simulink library "Batteries"  (R2026a)
settings: Solver=VariableStepAuto
undefined symbols (not defined in the file or in its folder): battery_builder_rtmsupport, gcbh
libraries: Batteries_lib x2
settings Model: Creator=dom  LastModifiedBy=dom

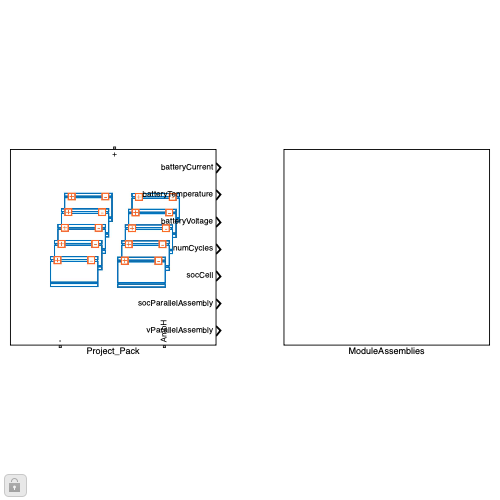
[thumbnail: Simulink's stored preview of the top-level diagram]
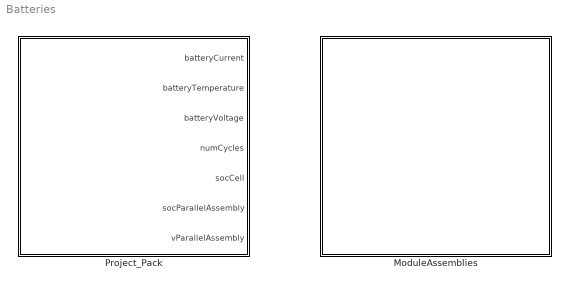
== system Batteries ==
  ModuleAssemblies : Subsystem
  Project_Pack : Subsystem  LoadFcn=battery_builder_rtmsupport('loadfcn',gcbh);
      settings: CopyFcn=battery_builder_rtmsupport('copyfcn',gcbh);  PreCopyFcn=battery_builder_rtmsupport('precopyfcn',gcbh);  PreDeleteFcn=battery_builder_rtmsupport('predeletefcn',gcbh);  PortSchema="{\"entries\":[{\"content\":{\"sides\":[{\"content\":{\"connectorIds\":[\"LConn1\"]},\"type\":\"ConnectorPlacement.EquallySpacedRectSide\",\"uuid\":\"76c6f046-db8e-4015-a922-00ba973faf16\"},{\"content\":{\"connectorIds\":[\"RConn1\",\"RConn2\"],\"side\":\"RIGHT\"},\"type\":\"ConnectorPlacement.EquallySpacedRectSide\",\"uuid\":\"59fdee5c-a6f4-4b44-aa6e-82d2d9418fce\"},{\"content\":{\"side\":\"TOP\"},\"type\":\"ConnectorPlacement.EquallySpacedRectSide\",\"uuid\":\"84b83595-cc1f-46da-a2b0-c16634a6daab\"},{\"content\":{\"connectorIds\":[\"Out1\",\"Out2\",\"Out3\",\"Out4\",\"Out5\",\"Out6\",\"Out7\"],\"side\":\"BOTTOM\"},\"type\":\"ConnectorPlacement.EquallySpacedRectSide\",\"uuid\":\"4528fa0d-8164-4e66-baa6-2a345765de4f\"}]},\"type\":\"ConnectorPlacement.EquallySpacedConnector\",\"uuid\":\"e6fb231a-8daf-4bfc-bdc1-9175fa7a2dfd\"}],\"packageUris\":[\"http://schema.mathworks.com/mf0/Connector/R2020b\"],\"version\":\"1.0\"}"
      mask Display: image('$imagefile')

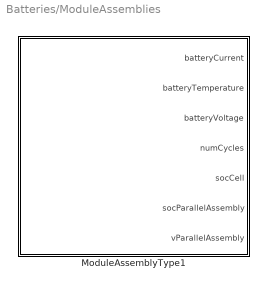
== system Batteries/ModuleAssemblies ==
  ModuleAssemblyType1 : Subsystem  LoadFcn=battery_builder_rtmsupport('loadfcn',gcbh);
      settings: CopyFcn=battery_builder_rtmsupport('copyfcn',gcbh);  PreCopyFcn=battery_builder_rtmsupport('precopyfcn',gcbh);  PreDeleteFcn=battery_builder_rtmsupport('predeletefcn',gcbh);  PortSchema="{\"entries\":[{\"content\":{\"sides\":[{\"content\":{\"connectorIds\":[\"LConn1\"]},\"type\":\"ConnectorPlacement.EquallySpacedRectSide\",\"uuid\":\"76c6f046-db8e-4015-a922-00ba973faf16\"},{\"content\":{\"connectorIds\":[\"RConn1\",\"RConn2\"],\"side\":\"RIGHT\"},\"type\":\"ConnectorPlacement.EquallySpacedRectSide\",\"uuid\":\"59fdee5c-a6f4-4b44-aa6e-82d2d9418fce\"},{\"content\":{\"side\":\"TOP\"},\"type\":\"ConnectorPlacement.EquallySpacedRectSide\",\"uuid\":\"84b83595-cc1f-46da-a2b0-c16634a6daab\"},{\"content\":{\"connectorIds\":[\"Out1\",\"Out2\",\"Out3\",\"Out4\",\"Out5\",\"Out6\",\"Out7\"],\"side\":\"BOTTOM\"},\"type\":\"ConnectorPlacement.EquallySpacedRectSide\",\"uuid\":\"391f6102-8f79-4306-a331-0bb83eeeb4a2\"}]},\"type\":\"ConnectorPlacement.EquallySpacedConnector\",\"uuid\":\"e6fb231a-8daf-4bfc-bdc1-9175fa7a2dfd\"}],\"packageUris\":[\"http://schema.mathworks.com/mf0/Connector/R2020b\"],\"version\":\"1.0\"}"
      mask Display: image('$imagefile')

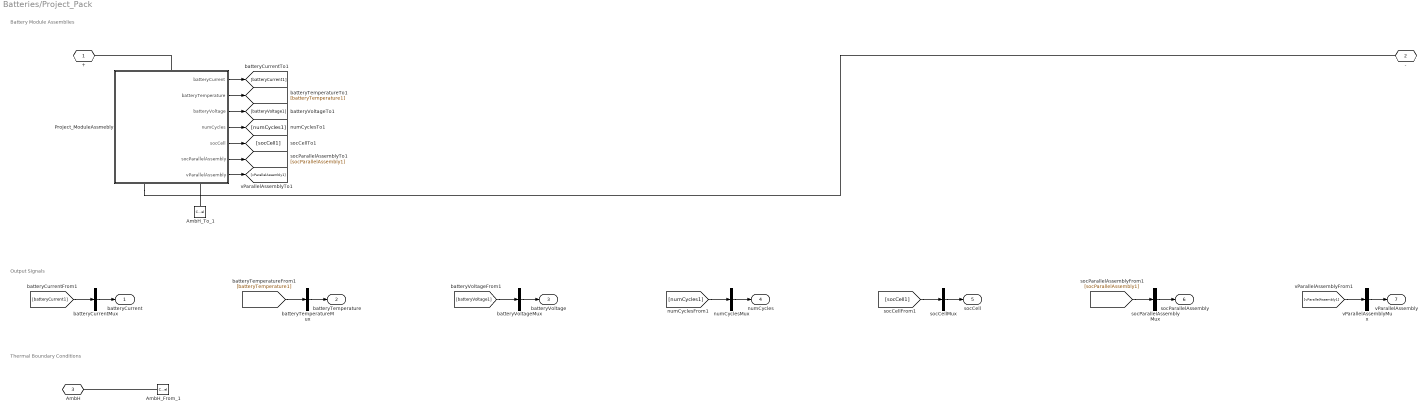
== system Batteries/Project_Pack ==
  note: Battery Module Assemblies
  note: Output Signals
  note: Thermal Boundary Conditions
  AmbH_From_1 : ConnectionLabel  Label=ambH_1
  AmbH_To_1 : ConnectionLabel  Label=ambH_1
  Project_ModuleAssmebly : Subsystem  LoadFcn=battery_builder_rtmsupport('loadfcn',gcbh);
      settings: CopyFcn=battery_builder_rtmsupport('copyfcn',gcbh);  PreCopyFcn=battery_builder_rtmsupport('precopyfcn',gcbh);  PreDeleteFcn=battery_builder_rtmsupport('predeletefcn',gcbh);  PortSchema="{\"entries\":[{\"content\":{\"sides\":[{\"content\":{\"connectorIds\":[\"LConn1\"]},\"type\":\"ConnectorPlacement.EquallySpacedRectSide\",\"uuid\":\"76c6f046-db8e-4015-a922-00ba973faf16\"},{\"content\":{\"connectorIds\":[\"RConn1\",\"RConn2\"],\"side\":\"RIGHT\"},\"type\":\"ConnectorPlacement.EquallySpacedRectSide\",\"uuid\":\"59fdee5c-a6f4-4b44-aa6e-82d2d9418fce\"},{\"content\":{\"side\":\"TOP\"},\"type\":\"ConnectorPlacement.EquallySpacedRectSide\",\"uuid\":\"84b83595-cc1f-46da-a2b0-c16634a6daab\"},{\"content\":{\"connectorIds\":[\"Out1\",\"Out2\",\"Out3\",\"Out4\",\"Out5\",\"Out6\",\"Out7\"],\"side\":\"BOTTOM\"},\"type\":\"ConnectorPlacement.EquallySpacedRectSide\",\"uuid\":\"391f6102-8f79-4306-a331-0bb83eeeb4a2\"}]},\"type\":\"ConnectorPlacement.EquallySpacedConnector\",\"uuid\":\"e6fb231a-8daf-4bfc-bdc1-9175fa7a2dfd\"}],\"packageUris\":[\"http://schema.mathworks.com/mf0/Connector/R2020b\"],\"version\":\"1.0\"}"
      mask Display: image('$imagefile')
  batteryCurrentMux : Mux  Inputs=1
  batteryTemperatureMux : Mux  Inputs=1
  batteryVoltageMux : Mux  Inputs=1
  numCyclesMux : Mux  Inputs=1
  socCellMux : Mux  Inputs=1
  socParallelAssemblyMux : Mux  Inputs=1
  vParallelAssemblyMux : Mux  Inputs=1
  + : PMIOPort  Side=Left
  - : PMIOPort  Port=2  Side=Right
  AmbH : PMIOPort  Port=3  Side=Right  ConnectionType=Connection: foundation.thermal.thermal
  batteryCurrent : Outport
  batteryTemperature : Outport  Port=2
  batteryVoltage : Outport  Port=3
  numCycles : Outport  Port=4
  socCell : Outport  Port=5
  socParallelAssembly : Outport  Port=6
  vParallelAssembly : Outport  Port=7
  wires:
  Project_ModuleAssmebly/1(batteryCurrent) -> [batteryCurrent1]
  batteryCurrentMux/1 -> batteryCurrent/1
  [batteryCurrent1] -> batteryCurrentMux/1
  Project_ModuleAssmebly/2(batteryTemperature) -> [batteryTemperature1]
  batteryTemperatureMux/1 -> batteryTemperature/1
  [batteryTemperature1] -> batteryTemperatureMux/1
  Project_ModuleAssmebly/3(batteryVoltage) -> [batteryVoltage1]
  batteryVoltageMux/1 -> batteryVoltage/1
  [batteryVoltage1] -> batteryVoltageMux/1
  Project_ModuleAssmebly/4(numCycles) -> [numCycles1]
  numCyclesMux/1 -> numCycles/1
  [numCycles1] -> numCyclesMux/1
  Project_ModuleAssmebly/5(socCell) -> [socCell1]
  socCellMux/1 -> socCell/1
  [socCell1] -> socCellMux/1
  Project_ModuleAssmebly/6(socParallelAssembly) -> [socParallelAssembly1]
  socParallelAssemblyMux/1 -> socParallelAssembly/1
  [socParallelAssembly1] -> socParallelAssemblyMux/1
  Project_ModuleAssmebly/7(vParallelAssembly) -> [vParallelAssembly1]
  vParallelAssemblyMux/1 -> vParallelAssembly/1
  [vParallelAssembly1] -> vParallelAssemblyMux/1
  connections:
  Project_ModuleAssmebly/LConn1 -- +/RConn1
  Project_ModuleAssmebly/RConn1 -- -/RConn1
  AmbH_To_1/LConn1 -- Project_ModuleAssmebly/RConn2
  AmbH_From_1/LConn1 -- AmbH/RConn1

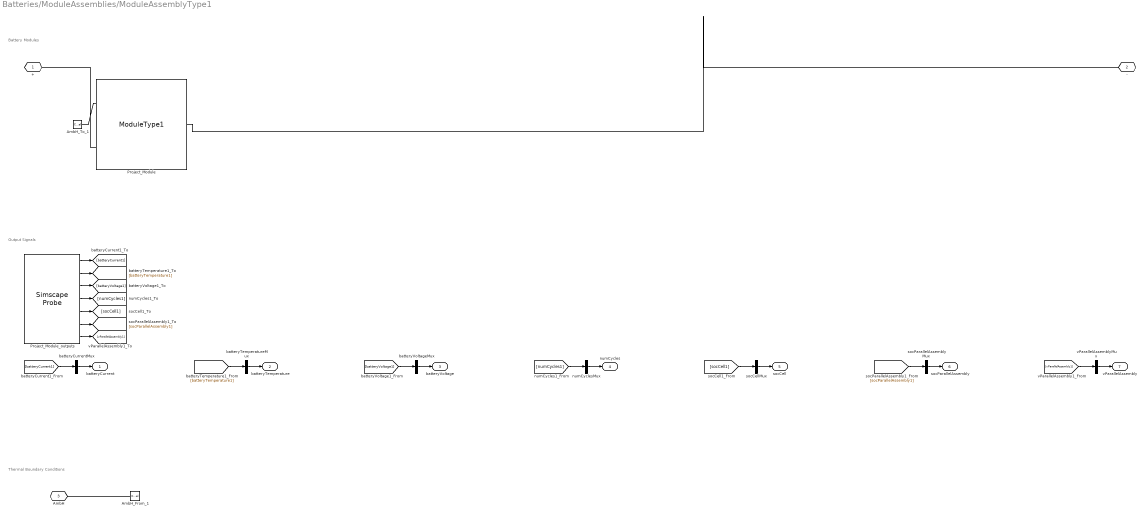
== system Batteries/ModuleAssemblies/ModuleAssemblyType1 ==
  note: Battery Modules
  note: Output Signals
  note: Thermal Boundary Conditions
  AmbH_From_1 : ConnectionLabel  Label=ambH_1
  AmbH_To_1 : ConnectionLabel  Label=ambH_1
  Project_Module : Batteries_lib/Modules/ModuleType1  BatteryCapacityCell=27 A*hr  ExtrapolationMethodCell=simscape.enum.extrapolation.nearest  SOCBreakpointsCell=[0, .1, .25, .5, .75, .9, 1]  TemperatureBreakpointsCell=[278, 293, 313] K  OpenCircuitVoltageThermalCell=[3.49, 3.5, 3.51; 3.55, 3.57, 3.56; 3.62, 3.63, 3.64; 3.71, 3.71, 3.72; 3.91, 3.93, 3.94; 4.07, 4.08, 4.08; 4.19, 4.19, 4.19] V  VoltageRangeCell=[0, inf] V  ResistanceSOCBreakpointsCell=[0, .1, .25, .5, .75, .9, 1]  ResistanceTemperatureBreakpointsCell=[278, 293, 313] K  R0ThermalCell=[.0117, .0085, .009; .011, .0085, .009; .0114, .0087, .0092; .0107, .0082, .0088; .0107, .0083, .0091; .0113, .0085, .0089; .0116, .0085, .0089] Ohm  BatteryThermalMassCell=100 J/K  AmbientResistance=25 K/W  socCell_specify=off  socCell_priority=High  socCell=1  socCell_nominal_specify=off  socCell_nominal_value=1  socCell_nominal_unit=1  batteryVoltage_specify=off  batteryVoltage_priority=None  batteryVoltage=0 V  batteryVoltage_nominal_specify=off  batteryVoltage_nominal_value=1  batteryVoltage_nominal_unit=V  batteryCurrent_specify=off  batteryCurrent_priority=None  batteryCurrent=0 A  batteryCurrent_nominal_specify=off  batteryCurrent_nominal_value=1  batteryCurrent_nominal_unit=A  numCycles_specify=off  numCycles_priority=High  numCycles=0  numCycles_nominal_specify=off  numCycles_nominal_value=1  numCycles_nominal_unit=1  batteryTemperature_specify=off  batteryTemperature_priority=High  batteryTemperature=298.15 K  batteryTemperature_nominal_specify=off  batteryTemperature_nominal_value=1  batteryTemperature_nominal_unit=K  vParallelAssembly_specify=off  vParallelAssembly_priority=None  vParallelAssembly=repmat(0, 10, 1) V  vParallelAssembly_nominal_specify=off  vParallelAssembly_nominal_value=1  vParallelAssembly_nominal_unit=V  socParallelAssembly_specify=off  socParallelAssembly_priority=None  socParallelAssembly=repmat(1, 10, 1)  socParallelAssembly_nominal_specify=off  socParallelAssembly_nominal_value=1  socParallelAssembly_nominal_unit=1
  Project_Module_outputs : SimscapeProbe  BoundBlock=3  Variables="{\"batteryCurrent\":{\"Probing\":\"ON\"},\"batteryTemperature\":{\"Probing\":\"ON\"},\"batteryVoltage\":{\"Probing\":\"ON\"},\"numCycles\":{\"Probing\":\"ON\"},\"socCell\":{\"Probing\":\"ON\"},\"socParallelAssembly\":{\"Probing\":\"ON\"},\"vParallelAssembly\":{\"Probing\":\"ON\"}}"
  batteryCurrentMux : Mux  Inputs=1
  batteryTemperatureMux : Mux  Inputs=1
  batteryVoltageMux : Mux  Inputs=1
  numCyclesMux : Mux  Inputs=1
  socCellMux : Mux  Inputs=1
  socParallelAssemblyMux : Mux  Inputs=1
  vParallelAssemblyMux : Mux  Inputs=1
  + : PMIOPort  Side=Left
  - : PMIOPort  Port=2  Side=Right
  AmbH : PMIOPort  Port=3  Side=Right  ConnectionType=Connection: foundation.thermal.thermal
  batteryCurrent : Outport
  batteryTemperature : Outport  Port=2
  batteryVoltage : Outport  Port=3
  numCycles : Outport  Port=4
  socCell : Outport  Port=5
  socParallelAssembly : Outport  Port=6
  vParallelAssembly : Outport  Port=7
  wires:
  Project_Module_outputs/1 -> [batteryCurrent1]
  batteryCurrentMux/1 -> batteryCurrent/1
  [batteryCurrent1] -> batteryCurrentMux/1
  Project_Module_outputs/2 -> [batteryTemperature1]
  batteryTemperatureMux/1 -> batteryTemperature/1
  [batteryTemperature1] -> batteryTemperatureMux/1
  Project_Module_outputs/3 -> [batteryVoltage1]
  batteryVoltageMux/1 -> batteryVoltage/1
  [batteryVoltage1] -> batteryVoltageMux/1
  Project_Module_outputs/4 -> [numCycles1]
  numCyclesMux/1 -> numCycles/1
  [numCycles1] -> numCyclesMux/1
  Project_Module_outputs/5 -> [socCell1]
  socCellMux/1 -> socCell/1
  [socCell1] -> socCellMux/1
  Project_Module_outputs/6 -> [socParallelAssembly1]
  socParallelAssemblyMux/1 -> socParallelAssembly/1
  [socParallelAssembly1] -> socParallelAssemblyMux/1
  Project_Module_outputs/7 -> [vParallelAssembly1]
  vParallelAssemblyMux/1 -> vParallelAssembly/1
  [vParallelAssembly1] -> vParallelAssemblyMux/1
  connections:
  Project_Module/LConn2 -- +/RConn1
  Project_Module/RConn1 -- -/RConn1
  AmbH_To_1/LConn1 -- Project_Module/LConn1
  AmbH_From_1/LConn1 -- AmbH/RConn1

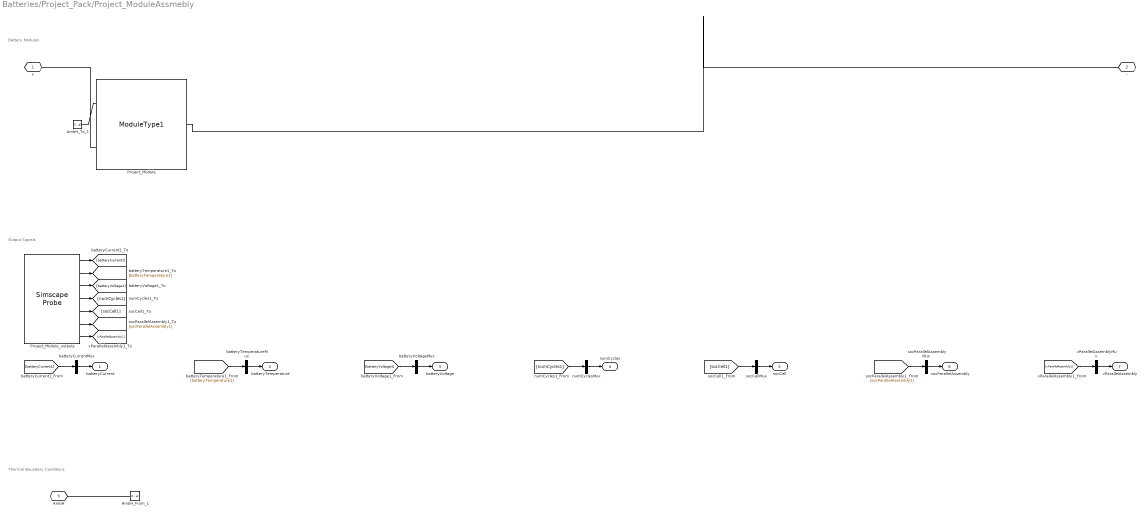
== system Batteries/Project_Pack/Project_ModuleAssmebly ==
  note: Thermal Boundary Conditions
  note: Output Signals
  note: Battery Modules
  AmbH_From_1 : ConnectionLabel  Label=ambH_1
  AmbH_To_1 : ConnectionLabel  Label=ambH_1
  Project_Module : Batteries_lib/Modules/ModuleType1  BatteryCapacityCell=27 A*hr  ExtrapolationMethodCell=simscape.enum.extrapolation.nearest  SOCBreakpointsCell=[0, .1, .25, .5, .75, .9, 1]  TemperatureBreakpointsCell=[278, 293, 313] K  OpenCircuitVoltageThermalCell=[3.49, 3.5, 3.51; 3.55, 3.57, 3.56; 3.62, 3.63, 3.64; 3.71, 3.71, 3.72; 3.91, 3.93, 3.94; 4.07, 4.08, 4.08; 4.19, 4.19, 4.19] V  VoltageRangeCell=[0, inf] V  ResistanceSOCBreakpointsCell=[0, .1, .25, .5, .75, .9, 1]  ResistanceTemperatureBreakpointsCell=[278, 293, 313] K  R0ThermalCell=[.0117, .0085, .009; .011, .0085, .009; .0114, .0087, .0092; .0107, .0082, .0088; .0107, .0083, .0091; .0113, .0085, .0089; .0116, .0085, .0089] Ohm  BatteryThermalMassCell=100 J/K  AmbientResistance=25 K/W  socCell_specify=off  socCell_priority=High  socCell=1  socCell_nominal_specify=off  socCell_nominal_value=1  socCell_nominal_unit=1  batteryVoltage_specify=off  batteryVoltage_priority=None  batteryVoltage=0 V  batteryVoltage_nominal_specify=off  batteryVoltage_nominal_value=1  batteryVoltage_nominal_unit=V  batteryCurrent_specify=off  batteryCurrent_priority=None  batteryCurrent=0 A  batteryCurrent_nominal_specify=off  batteryCurrent_nominal_value=1  batteryCurrent_nominal_unit=A  numCycles_specify=off  numCycles_priority=High  numCycles=0  numCycles_nominal_specify=off  numCycles_nominal_value=1  numCycles_nominal_unit=1  batteryTemperature_specify=off  batteryTemperature_priority=High  batteryTemperature=298.15 K  batteryTemperature_nominal_specify=off  batteryTemperature_nominal_value=1  batteryTemperature_nominal_unit=K  vParallelAssembly_specify=off  vParallelAssembly_priority=None  vParallelAssembly=repmat(0, 10, 1) V  vParallelAssembly_nominal_specify=off  vParallelAssembly_nominal_value=1  vParallelAssembly_nominal_unit=V  socParallelAssembly_specify=off  socParallelAssembly_priority=None  socParallelAssembly=repmat(1, 10, 1)  socParallelAssembly_nominal_specify=off  socParallelAssembly_nominal_value=1  socParallelAssembly_nominal_unit=1
  Project_Module_outputs : SimscapeProbe  BoundBlock=45  Variables="{\"batteryCurrent\":{\"Probing\":\"ON\"},\"batteryTemperature\":{\"Probing\":\"ON\"},\"batteryVoltage\":{\"Probing\":\"ON\"},\"numCycles\":{\"Probing\":\"ON\"},\"socCell\":{\"Probing\":\"ON\"},\"socParallelAssembly\":{\"Probing\":\"ON\"},\"vParallelAssembly\":{\"Probing\":\"ON\"}}"
  batteryCurrentMux : Mux  Inputs=1
  batteryTemperatureMux : Mux  Inputs=1
  batteryVoltageMux : Mux  Inputs=1
  numCyclesMux : Mux  Inputs=1
  socCellMux : Mux  Inputs=1
  socParallelAssemblyMux : Mux  Inputs=1
  vParallelAssemblyMux : Mux  Inputs=1
  + : PMIOPort  Side=Left
  - : PMIOPort  Port=2  Side=Right
  AmbH : PMIOPort  Port=3  Side=Right  ConnectionType=Connection: foundation.thermal.thermal
  batteryCurrent : Outport
  batteryTemperature : Outport  Port=2
  batteryVoltage : Outport  Port=3
  numCycles : Outport  Port=4
  socCell : Outport  Port=5
  socParallelAssembly : Outport  Port=6
  vParallelAssembly : Outport  Port=7
  wires:
  [vParallelAssembly1] -> vParallelAssemblyMux/1
  vParallelAssemblyMux/1 -> vParallelAssembly/1
  Project_Module_outputs/7 -> [vParallelAssembly1]
  [socParallelAssembly1] -> socParallelAssemblyMux/1
  socParallelAssemblyMux/1 -> socParallelAssembly/1
  Project_Module_outputs/6 -> [socParallelAssembly1]
  [socCell1] -> socCellMux/1
  socCellMux/1 -> socCell/1
  Project_Module_outputs/5 -> [socCell1]
  [numCycles1] -> numCyclesMux/1
  numCyclesMux/1 -> numCycles/1
  Project_Module_outputs/4 -> [numCycles1]
  [batteryVoltage1] -> batteryVoltageMux/1
  batteryVoltageMux/1 -> batteryVoltage/1
  Project_Module_outputs/3 -> [batteryVoltage1]
  [batteryTemperature1] -> batteryTemperatureMux/1
  batteryTemperatureMux/1 -> batteryTemperature/1
  Project_Module_outputs/2 -> [batteryTemperature1]
  [batteryCurrent1] -> batteryCurrentMux/1
  batteryCurrentMux/1 -> batteryCurrent/1
  Project_Module_outputs/1 -> [batteryCurrent1]
  connections:
  AmbH_From_1/LConn1 -- AmbH/RConn1
  AmbH_To_1/LConn1 -- Project_Module/LConn1
  Project_Module/RConn1 -- -/RConn1
  Project_Module/LConn2 -- +/RConn1
